simulink subsystem "DutyCycle2_Level"  (R2024b)
settings: Solver=VariableStepAuto  StartTime=0.0  StopTime=10.0  RelTol=1e-3
settings Model: Creator=rodri  LastModifiedBy=rodri
settings RTWCC: GPUComputeCapability=3.5

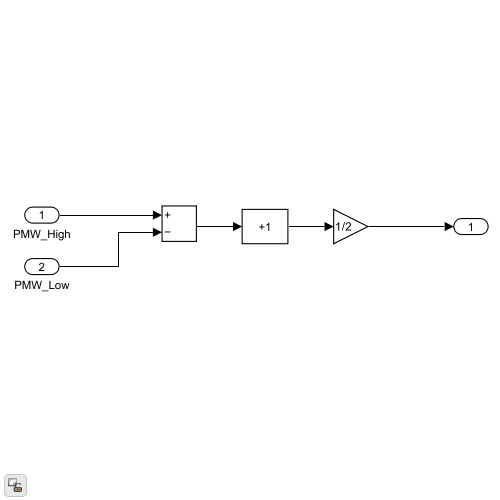
[thumbnail: Simulink's stored preview of the top-level diagram]
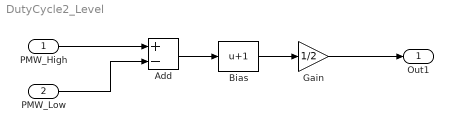
== system DutyCycle2_Level ==
  PMW_High : Inport
  PMW_Low : Inport  Port=2
  Add : Sum  Inputs=+-
  Bias : Bias  Bias=1  SaturateOnIntegerOverflow=off
  Gain : Gain  Gain=1/2
  Out1 : Outport  OutMin=0  OutMax=1
  wires:
  PMW_High/1 -> Add/1
  Add/1 -> Bias/1
  PMW_Low/1 -> Add/2
  Bias/1 -> Gain/1
  Gain/1 -> Out1/1
